simulink model "commhdlQPSKTxRxLoopback"  (R2025b)
settings: Solver=FixedStepDiscrete  StartTime=0.0  StopTime=0.03  RelTol=1e-3
PostLoadFcn:
  | hScopeConfig = get_param([gcs '/Receiver/QPSK Rx/Frequency and Time Synchronizer/Symbol Synchronizer/No HDL/QPSK Receiver Eye Diagram'],'ScopeConfiguration');
  | 
  | hScopeConfig.OpenAtSimulationStart = false;
  | hScopeConfig.Visible = false;
  | SamplesPerSymbol = 4;
  | %UpsamplesRx = 1;
  | clear hScopeConfig
InitFcn:
  | % RxAlign decoder latency (flat_simfix): 41 = netlist value used for HDL; set
  | % rxAlignLat = 25 in the base workspace before a model-level simulation.
  | if ~exist('rxAlignLat','var'), rxAlignLat = uint16(41); end
  | commhdlQPSKTxRxModelInit;
  | % Rate bridge: ADRV9002/Jupiter radio runs at 15.36 MHz = 2x the 7.68 MHz
  | % (4 samples/symbol @ Rsym=1.92 MHz) the QPSK Rx requires. The deployed
  | % Receiver must downsample the ADC stream by 2. UpsamplesRx=1 fed the QPSK
  | % Rx 8 sps (2x-upsampled) and broke symbol sync / the loopback bit check.
  | UpsamplesRx = 1;   %% T8 RATE FIX: rail 15.36e6 == ADC bus rate,
  | %% no ingress decimation (was 2 when the rail sat on the 7.68e6 rung)
  | UpsamplesTx = 1;
  | clear simTimingOffset;
StopFcn:
  | if exist('simTimingOffset','var')
  |   disp('Simulation completed');
  |   %QPSKTxRxVerification;
  | end
undefined symbols (not defined in the file or in its folder): Add, Config, fsym, randsrc, RandStream, Rsym, rxAlignLat, Shift
libraries: hdlsllib x141, simulink x45, dspsigops x30, dsphdlfiltering2 x6, dsphdlsigops2 x4, dsphdlmathfun2 x4, commdigbbndpm3 x4, dspmlti4 x2, commchan3 x1, commrflib2 x1, commcnvcod2 x1
(part 3 of 9)

== system commhdlQPSKTxRxLoopback/Transmitter/Input Data/Message Generator ==
  reset : Inport
  enable : Inport  Port=2
  MATLAB Function : MATLAB Function  TreatAsAtomicUnit=on
  out : Outport
  stop : Outport  Port=2
  start : Outport  Port=3
  valid : Outport  Port=4
  count : Outport  Port=5
  msg_count_out : Outport  Port=6
  wires:
  MATLAB Function/3(stop) -> stop/1
  MATLAB Function/1(out) -> out/1
  reset/1 -> MATLAB Function/2(reset)
  MATLAB Function/2(start) -> start/1
  enable/1 -> MATLAB Function/1(enable)
  MATLAB Function/4(valid) -> valid/1
  MATLAB Function/5(count_out) -> count/1
  MATLAB Function/6(msg_count_out) -> msg_count_out/1

== system commhdlQPSKTxRxLoopback/Transmitter/QPSK Tx/Bit Packetizer ==
  dataIn : Inport
  validIn : Inport  Port=2
  Compare To Constant : hdlsllib/Logic and Bit Operations/Compare To Constant  relop===  const=length(Preamble)  OutDataTypeStr=boolean
  Compare To Constant1 : hdlsllib/Logic and Bit Operations/Compare To Constant  relop===  const=bitsPerPacket - 1  OutDataTypeStr=boolean
  Compare To Constant2 : hdlsllib/Logic and Bit Operations/Compare To Constant  relop=>=  const=length(Preamble)  OutDataTypeStr=boolean
  Data Bits FIFO : Subsystem
  Data Type Conversion : DataTypeConversion  OutDataTypeStr=boolean  SaturateOnIntegerOverflow=off  RndMeth=Floor
  DataReadyPaceCmp : simulink/Logic and Bit Operations/Compare To Constant  relop=>=  const=SamplesPerSymbol/2 - 1  OutDataTypeStr=boolean
  HDL Counter : hdlsllib/Sources/HDL Counter  CountType=Count limited  CountInit=0  CountStep=1  CountMax=max(1, SamplesPerSymbol/2 - 1)  CountFromType=Initial value  CountFrom=0  CountResetPort=off  CountLoadPort=off  CountEnbPort=on  CountDirPort=off  CountHitOutputPort=off  CountDataType=Unsigned  CountWordLen=max(1, nextpow2(SamplesPerSymbol/2))  CountFracLen=0  CountSampTime=1
  Logical Operator : Logic  AllPortsSameDT=off  OutDataTypeStr=boolean
  Logical Operator1 : Logic  AllPortsSameDT=off  OutDataTypeStr=boolean
  Logical Operator2 : Logic  Operator=NOT  AllPortsSameDT=off  OutDataTypeStr=boolean
  Preamble Bits Generator : Subsystem
  Switch : Switch  Criteria=u2 ~= 0  SaturateOnIntegerOverflow=off  InputSameDT=off
  bitsOut : Outport
  dataStart : Outport  Port=2
  dataEnd : Outport  Port=3
  bitsValid : Outport  Port=4
  dataReady : Outport  Port=5
  wires:
  dataIn/1 -> Data Bits FIFO/1(data)
  validIn/1 -> Data Bits FIFO/2(push)
  Compare To Constant/1 -> Logical Operator/1
  Compare To Constant1/1 -> Logical Operator1/2
  Logical Operator/1 -> dataStart/1
  Logical Operator1/1 -> dataEnd/1
  Data Bits FIFO/5(fullRAM) -> Logical Operator2/1
  Logical Operator2/1 -> HDL Counter/1
  Data Bits FIFO/1(dataOut) -> Switch/1
  Data Bits FIFO/3(sampleCount) -> Preamble Bits Generator/2(sampleCount), Compare To Constant/1, Compare To Constant1/1, Compare To Constant2/1
  Data Bits FIFO/4(sampleCountValid) -> bitsValid/1, Logical Operator/2, Logical Operator1/1, Preamble Bits Generator/3(sampleCountValid)
  Data Bits FIFO/2(activeFrame) -> Preamble Bits Generator/1(activeFrame)
  Preamble Bits Generator/1(preambleBits) -> Switch/3
  Compare To Constant2/1 -> Switch/2
  Switch/1 -> bitsOut/1
  Data Type Conversion/1 -> dataReady/1
  HDL Counter/1 -> DataReadyPaceCmp/1
  DataReadyPaceCmp/1 -> Data Type Conversion/1

== system commhdlQPSKTxRxLoopback/Transmitter/QPSK Tx/HDL Data Scrambler ==
  note: HDL Data Scrambler
      | Polynomial: x^7+x^4+1
      | Initial state: [1 0 1 1 1 0 1]
  dataIn : Inport
  startIn : Inport  Port=2
  endIn : Inport  Port=3
  validIn : Inport  Port=4
  BIT_XOR : Logic  Operator=XOR  IconShape=distinctive  AllPortsSameDT=off  OutDataTypeStr=boolean
  BIT_XOR2 : Logic  Operator=XOR  IconShape=distinctive  AllPortsSameDT=off  OutDataTypeStr=boolean
  Delay{,1,3..4} (4 alike) : Delay  DelayLength=1
  EnableScrambling : Constant  Value=true  SampleTime=-1
  Logical Operator : Logic  IconShape=distinctive  AllPortsSameDT=off  OutDataTypeStr=boolean
  Switch : Switch  Criteria=u2 > Threshold  SaturateOnIntegerOverflow=off  InputSameDT=off
  Unit Delay Enabled Resettable Synchronous{,2..3,5,7} (5 alike) : hdlsllib/Discrete/Unit Delay Enabled Resettable Synchronous  InitialCondition=1  SampleTime=-1
  Unit Delay Enabled Resettable Synchronous1 : hdlsllib/Discrete/Unit Delay Enabled Resettable Synchronous  InitialCondition=0  SampleTime=-1
  Unit Delay Enabled Resettable Synchronous4 : hdlsllib/Discrete/Unit Delay Enabled Resettable Synchronous  InitialCondition=0  SampleTime=-1
  Unit Delay Enabled Resettable Synchronous6 : hdlsllib/Discrete/Unit Delay Enabled Resettable Synchronous  InitialCondition=0.0  SampleTime=-1
  dataOut : Outport  InitialOutput=0
  validOut : Outport  Port=2  InitialOutput=0
  wires:
  Delay4/1 -> validOut/1
  Delay3/1 -> dataOut/1
  endIn/1 -> Unit Delay Enabled Resettable Synchronous4/3
  Logical Operator/1 -> BIT_XOR2/2
  Unit Delay Enabled Resettable Synchronous4/1 -> Logical Operator/1
  Delay1/1 -> Unit Delay Enabled Resettable Synchronous6/2, Unit Delay Enabled Resettable Synchronous2/2, Unit Delay Enabled Resettable Synchronous1/2, Unit Delay Enabled Resettable Synchronous/2, Delay4/1, Unit Delay Enabled Resettable Synchronous3/2, Unit Delay Enabled Resettable Synchronous5/2, Unit Delay Enabled Resettable Synchronous7/2
  Delay/1 -> Switch/3, BIT_XOR2/1
  startIn/1 -> Unit Delay Enabled Resettable Synchronous4/1, Unit Delay Enabled Resettable Synchronous4/2, Unit Delay Enabled Resettable Synchronous6/3, Unit Delay Enabled Resettable Synchronous5/3, Unit Delay Enabled Resettable Synchronous1/3, Unit Delay Enabled Resettable Synchronous/3, Unit Delay Enabled Resettable Synchronous2/3, Unit Delay Enabled Resettable Synchronous3/3, Unit Delay Enabled Resettable Synchronous7/3
  dataIn/1 -> Delay/1
  validIn/1 -> Delay1/1
  BIT_XOR/1 -> Unit Delay Enabled Resettable Synchronous/1, Logical Operator/2
  Unit Delay Enabled Resettable Synchronous1/1 -> Unit Delay Enabled Resettable Synchronous2/1
  Unit Delay Enabled Resettable Synchronous2/1 -> Unit Delay Enabled Resettable Synchronous3/1
  Unit Delay Enabled Resettable Synchronous/1 -> Unit Delay Enabled Resettable Synchronous1/1
  Unit Delay Enabled Resettable Synchronous3/1 -> BIT_XOR/2, Unit Delay Enabled Resettable Synchronous5/1
  Unit Delay Enabled Resettable Synchronous5/1 -> Unit Delay Enabled Resettable Synchronous6/1
  Unit Delay Enabled Resettable Synchronous6/1 -> Unit Delay Enabled Resettable Synchronous7/1
  Unit Delay Enabled Resettable Synchronous7/1 -> BIT_XOR/1
  Switch/1 -> Delay3/1
  EnableScrambling/1 -> Switch/2
  BIT_XOR2/1 -> Switch/1

== system commhdlQPSKTxRxLoopback/Transmitter/QPSK Tx/QPSK Modulator ==
  dataIn : Inport
  validIn : Inport  Port=2
  Compare To Constant : simulink/Logic and Bit Operations/Compare To Constant  relop===  const=0  OutDataTypeStr=boolean
  Compare To Constant1 : simulink/Logic and Bit Operations/Compare To Constant  relop===  const=1  OutDataTypeStr=boolean
  Delay{,1..5,11..12} (8 alike) : Delay  DelayLength=1
  HDL Counter : hdlsllib/Sources/HDL Counter  CountType=Count limited  CountInit=0  CountStep=1  CountMax=1  CountFromType=Initial value  CountFrom=0  CountResetPort=off  CountLoadPort=off  CountEnbPort=on  CountDirPort=off  CountHitOutputPort=off  CountDataType=Unsigned  CountWordLen=1  CountFracLen=0  CountSampTime=1
  Logical Operator : Logic  IconShape=distinctive  AllPortsSameDT=off  OutDataTypeStr=boolean
  Logical Operator1 : Logic  IconShape=distinctive  AllPortsSameDT=off  OutDataTypeStr=boolean
  Mux : Mux  Inputs=2
  Null : Constant  Value=complex(0,0)  OutDataTypeStr=fixdt(1,16,15)  SampleTime=1/(Rsym*SamplesPerSymbol)
  QPSK Modulator Baseband : commdigbbndpm3/QPSK Modulator Baseband  InType=Bit  Enc=Gray  Ph=pi/4  outDtype=Fixed-point  outWordLen=16  outUDDataType=sfix(16)  outFracLenMode=User-defined  outFracLen=15  outDataTypeStr=fixdt(1,16,15)  outLastDataTypeStr=fixdt(1,16,15)
  Switch3 : Switch  Threshold=1  SaturateOnIntegerOverflow=off  InputSameDT=off
  Unit Delay Enabled Synchronous : hdlsllib/Discrete/Unit Delay Enabled Synchronous  InitialCondition=0.0  SampleTime=-1
  dataOut : Outport
  validOut : Outport  Port=2
  wires:
  dataIn/1 -> Delay/1
  validIn/1 -> Delay1/1
  HDL Counter/1 -> Compare To Constant/1, Compare To Constant1/1
  QPSK Modulator Baseband/1 -> Delay11/1
  Logical Operator1/1 -> Delay5/1
  Switch3/1 -> Delay2/1
  Null/1 -> Switch3/3
  Delay/1 -> Mux/2, Unit Delay Enabled Synchronous/1
  Delay2/1 -> dataOut/1
  Delay3/1 -> validOut/1
  Delay1/1 -> Logical Operator1/2, Logical Operator/1, HDL Counter/1
  Compare To Constant/1 -> Logical Operator/2
  Compare To Constant1/1 -> Logical Operator1/1
  Delay11/1 -> Switch3/1
  Delay12/1 -> Switch3/2, Delay3/1
  Logical Operator/1 -> Unit Delay Enabled Synchronous/2
  Unit Delay Enabled Synchronous/1 -> Mux/1
  Mux/1 -> Delay4/1
  Delay4/1 -> QPSK Modulator Baseband/1
  Delay5/1 -> Delay12/1

== system commhdlQPSKTxRxLoopback/Transmitter/QPSK Tx/RRC Transmit Filter ==
  dataIn : Inport
  validIn : Inport  Port=2
  Data Type Conversion : DataTypeConversion  OutDataTypeStr=fixdt(1,17,16)  SaturateOnIntegerOverflow=off  RndMeth=Floor
  Data Type Conversion1 : DataTypeConversion  OutDataTypeStr=fixdt(1,16,14)  SaturateOnIntegerOverflow=off  RndMeth=Floor
  Delay1 : Delay  DelayLength=1
  Delay2 : Delay  DelayLength=1
  Delay3 : Delay  DelayLength=1
  RRC Filter : dsphdlfiltering2/Discrete FIR Filter  NumeratorSource=Property  Numerator=RRCCoef  NumeratorPrototype=[]  FilterStructure=Direct form systolic  SerializationOption=Minimum number of cycles between valid input samples  NumCycles=2  NumberOfMultipliers=2  SimulateUsing=Code generation  roundingMode=Floor  overflowMode=off  CoefficientsDataTypeStr=Inherit: Same word length as input  OutputDataTypeStr=Inherit: Same word length as input  ResetInputPort=off  HDLGlobalReset=off  CoeffMultiplier=Multiplier  UseMultForPow2Coeff=on  FrameInputSymmOptim=off
  Unit Delay Enabled Synchronous1 : hdlsllib/Discrete/Unit Delay Enabled Synchronous  InitialCondition=0  SampleTime=-1
  dataOut : Outport
  validOut : Outport  Port=2
  wires:
  dataIn/1 -> Data Type Conversion/1
  RRC Filter/1 -> Data Type Conversion1/1
  RRC Filter/2 -> Delay2/1
  Delay1/1 -> dataOut/1
  Delay2/1 -> validOut/1
  Data Type Conversion/1 -> Delay3/1
  Unit Delay Enabled Synchronous1/1 -> RRC Filter/2
  Data Type Conversion1/1 -> Delay1/1
  validIn/1 -> Unit Delay Enabled Synchronous1/2, Unit Delay Enabled Synchronous1/1
  Delay3/1 -> RRC Filter/1

== system commhdlQPSKTxRxLoopback/TxRxComposite/Receiver/Capture Data Bits ==
  dataOut : Inport
  dataSrt : Inport  Port=2
  dataEnd : Inport  Port=3
  valid : Inport  Port=4
  Display : Display
  Display1 : Display
  Display2 : Display
  MATLAB Function : MATLAB Function  TreatAsAtomicUnit=on
  count_out : Outport
  packets_out : Outport  Port=2
  bit_errors_out : Outport  Port=3
  wires:
  MATLAB Function/3(bit_errors_out) -> bit_errors_out/1, Display2/1
  MATLAB Function/2(packets_out) -> packets_out/1, Display1/1
  valid/1 -> MATLAB Function/1(valid)
  dataSrt/1 -> MATLAB Function/3(start)
  MATLAB Function/1(count_out) -> count_out/1, Display/1
  dataEnd/1 -> MATLAB Function/4(stop)
  dataOut/1 -> MATLAB Function/2(datain)

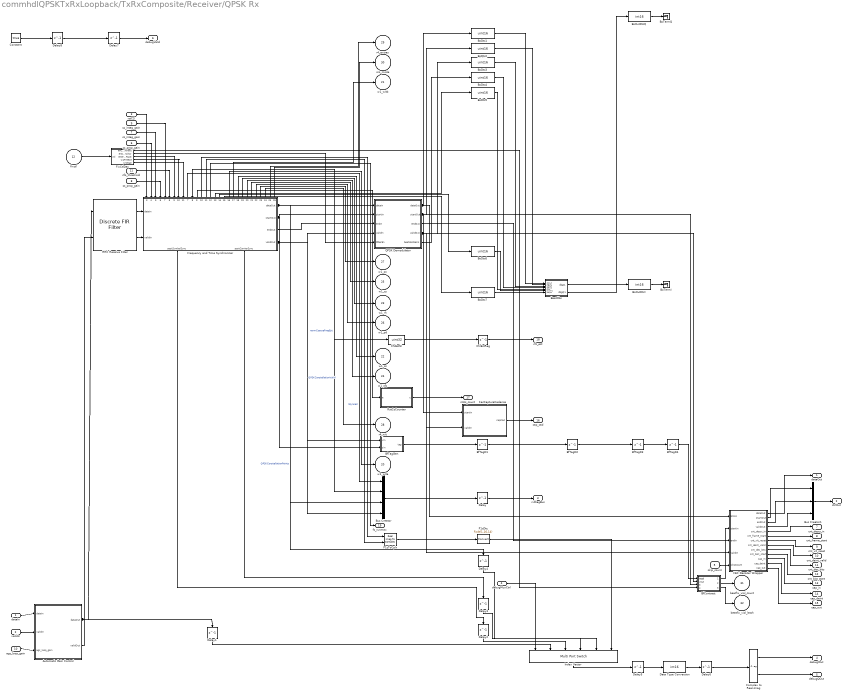
== system commhdlQPSKTxRxLoopback/TxRxComposite/Receiver/QPSK Rx ==
  dataIn : Inport  OutDataTypeStr=fixdt(1,16,14)  PortDimensions=1  SampleTime=1/(Rsym*SamplesPerSymbol)
      settings: SignalType=complex
  validIn : Inport  Port=2  OutDataTypeStr=boolean  PortDimensions=1  SampleTime=1/(Rsym*SamplesPerSymbol)
  rstCS : Inport  Port=3  OutDataTypeStr=boolean  PortDimensions=1
      settings: SignalType=complex
  debugMuxCtrl : Inport  Port=4  OutDataTypeStr=uint32  PortDimensions=1  SampleTime=1/(Rsym*SamplesPerSymbol)
  skip_count : Inport  Port=5  OutDataTypeStr=uint32  SampleTime=1/(Rsym*SamplesPerSymbol)
  cs_prop_gain : Inport  Port=6  OutDataTypeStr=uint32  SampleTime=1/(Rsym*SamplesPerSymbol)
  cs_integ_gain : Inport  Port=7  OutDataTypeStr=uint32  SampleTime=1/(Rsym*SamplesPerSymbol)
  ss_prop_gain : Inport  Port=8  OutDataTypeStr=uint32  SampleTime=1/(Rsym*SamplesPerSymbol)
  ss_integ_gain : Inport  Port=9  OutDataTypeStr=uint32  SampleTime=1/(Rsym*SamplesPerSymbol)
  agc_loop_gain : Inport  Port=10  OutDataTypeStr=uint32  SampleTime=1/(Rsym*SamplesPerSymbol)
  cfo_threshold : Inport  Port=11  OutDataTypeStr=uint32  SampleTime=1/(Rsym*SamplesPerSymbol)
  fixctl : Inport  Port=12  OutDataTypeStr=uint32
  Automatic Gain Control : Subsystem  mask{Ref=AGCReference, LFG=AGCLoopGain}
      mask prompts: Ref "Error Detector Reference:"; LFG "Loop Filter Gain"
  BeatObs : MATLAB Function  TreatAsAtomicUnit=on
  BfContract : MATLAB Function  TreatAsAtomicUnit=on
  BfTagD{1..4} (4 alike) : Delay  DelayLength=1
  BfTagGen : MATLAB Function  TreatAsAtomicUnit=on
  BoDtc{1..7} (7 alike) : DataTypeConversion  OutDataTypeStr=uint16  ConvertRealWorld=Stored Integer (SI)  SaturateOnIntegerOverflow=off  RndMeth=Floor
  BoOutDtcI : DataTypeConversion  OutDataTypeStr=int16  ConvertRealWorld=Stored Integer (SI)  SaturateOnIntegerOverflow=off  RndMeth=Floor
  BoOutDtcQ : DataTypeConversion  OutDataTypeStr=int16  ConvertRealWorld=Stored Integer (SI)  SaturateOnIntegerOverflow=off  RndMeth=Floor
  BoTermI : Terminator
  BoTermQ : Terminator
  Bus Creator : BusCreator  Inputs=4
  Bus Creator1 : BusCreator  Inputs=3
  CfcEstReg : Delay  DelayLength=1
  CfcEstSI : DataTypeConversion  OutDataTypeStr=uint32  ConvertRealWorld=Stored Integer (SI)
  Complex to Real-Imag : ComplexToRealImag
  Constant : Constant  Value=true  SampleTime=1/(Rsym*SamplesPerSymbol)
  Data Type Conversion : DataTypeConversion  OutDataTypeStr=int16  ConvertRealWorld=Stored Integer (SI)  SaturateOnIntegerOverflow=off  RndMeth=Floor
  Delay{,1..8} (9 alike) : Delay  DelayLength=1
  FEC Decoder Wrapper : Subsystem
  FecCaptureCadence : MATLAB Function  TreatAsAtomicUnit=on
  FixCtlDec : MATLAB Function  TreatAsAtomicUnit=on
  Frequency and Time Synchronizer : Subsystem
      settings: PortSchema="{\"entries\":[{\"content\":{\"sides\":[{\"content\":{\"connectorIds\":[\"In1\",\"In2\"]},\"type\":\"ConnectorPlacement.EquallySpacedRectSide\",\"uuid\":\"8bc6a452-5111-4806-8ca9-335cb622aea6\"},{\"content\":{\"connectorIds\":[\"Out1\",\"Out2\",\"Out3\",\"Out4\"],\"side\":\"RIGHT\"},\"type\":\"ConnectorPlacement.EquallySpacedRectSide\",\"uuid\":\"b0f43c98-f5c0-4f62-94ae-d69789942eef\"},{\"content\":{\"connectorIds\":[\"In3\",\"In4\",\"In5\",\"In6\",\"In7\",\"In8\",\"In9\",\"In10\",\"In11\",\"Out7\",\"Out8\",\"Out9\",\"Out10\",\"Out11\",\"Out12\",\"Out13\",\"Out14\",\"Out15\",\"Out16\",\"Out17\",\"Out18\",\"Out19\",\"Out20\",\"Out21\",\"Out22\",\"Out23\",\"Out24\",\"Out25\",\"Out26\"],\"side\":\"TOP\"},\"type\":\"ConnectorPlacement.EquallySpacedRectSide\",\"uuid\":\"427ff3b3-b896-4008-9584-d311480df763\"},{\"content\":{\"connectorIds\":[\"Out5\",\"Out6\"],\"side\":\"BOTTOM\"},\"type\":\"ConnectorPlacement.EquallySpacedRectSide\",\"uuid\":\"f704cb90-80a1-4198-8b72-e70182b45e73\"},{\"content\":{\"side\":\"HIDDEN\"},\"type\":\"ConnectorPlacement.EquallySpacedRectSide\",\"uuid\":\"f6309498-1e43-486f-b6b5-2c6570711f8e\"}]},\"type\":\"ConnectorPlacement.EquallySpacedConnector\",\"uuid\":\"f0ce492e-c9e1-4b35-98ef-84d77b696cfe\"}],\"packageUris\":[\"http://schema.mathworks.com/mf0/Connector/R2020b\"],\"version\":\"1.0\"}"
  Index Vector : MultiPortSwitch  DataPortOrder=Zero-based contiguous  Inputs=5  DiagnosticForDefault=None  zeroidx=on  SaturateOnIntegerOverflow=off  InputSameDT=off
  P1cDtc : DataTypeConversion  OutDataTypeStr=fixdt(1,16,14)  ConvertRealWorld=Stored Integer (SI)  SaturateOnIntegerOverflow=off  RndMeth=Floor
  P1cToCplx : RealImagToComplex
  QPSK Demodulator : Subsystem
  RRC Receive Filter : dsphdlfiltering2/Discrete FIR Filter  NumeratorSource=Property  Numerator=RRCCoef  NumeratorPrototype=[]  FilterStructure=Direct form systolic  SerializationOption=Minimum number of cycles between valid input samples  NumCycles=2  NumberOfMultipliers=2  SimulateUsing=Code generation  roundingMode=Floor  overflowMode=off  CoefficientsDataTypeStr=Inherit: Same word length as input  OutputDataTypeStr=Inherit: Same word length as input  ResetInputPort=off  HDLGlobalReset=off  CoeffMultiplier=Multiplier  UseMultForPow2Coeff=on  FrameInputSymmOptim=off
  RstCsCounter : MATLAB Function  TreatAsAtomicUnit=on
  dataOut : Outport
  ctrlOut : Outport  Port=2
  rxDiagBus : Outport  Port=3
  debugIOut : Outport  Port=4
  debugQOut : Outport  Port=5
  debugValid : Outport  Port=6
  cnt_descr_in : Outport  Port=7
  cnt_frame_start : Outport  Port=8
  cnt_vit_reset : Outport  Port=9
  cnt_deint_valid : Outport  Port=10
  cnt_dec_bits : Outport  Port=11
  cnt_bist_start : Outport  Port=12
  cap_in : Outport  Port=13
  cap_deint : Outport  Port=14
  cap_out : Outport  Port=15
  cap_cad : Outport  Port=16
  rstcs_count : Outport  Port=17
  cfc_est : Outport  Port=18
  fs_runmax : Outport  Port=19
  w1_wita : Outport  Port=20
  w1_witb : Outport  Port=21
  w1_ss : Outport  Port=22
  w1_rh : Outport  Port=23
  w1_cfc : Outport  Port=24
  w1_cs : Outport  Port=25
  w1_pd : Outport  Port=26
  w1_pc : Outport  Port=27
  r4_wit : Outport  Port=28
  r4_extras : Outport  Port=29
  sro_mode : Outport  Port=30
  beatfix_viol_count : Outport  Port=31
  beatfix_viol_latch : Outport  Port=32
  wires:
  Bus Creator1/1 -> ctrlOut/1
  FEC Decoder Wrapper/10(cnt_bist_start) -> cnt_bist_start/1
  FEC Decoder Wrapper/8(cnt_deint_valid) -> cnt_deint_valid/1
  FEC Decoder Wrapper/7(cnt_vit_reset) -> cnt_vit_reset/1
  FEC Decoder Wrapper/5(cnt_descr_in) -> cnt_descr_in/1
  Complex to Real-Imag/2 -> debugQOut/1
  FEC Decoder Wrapper/3(endOut) -> Bus Creator1/2
  FEC Decoder Wrapper/9(cnt_dec_bits) -> cnt_dec_bits/1
  skip_count/1 -> FEC Decoder Wrapper/5(skipCount)
  Delay5/1 -> Data Type Conversion/1
  BoOutDtcI/1 -> BoTermI/1
  BfTagD2/1 -> BfTagD3/1
  debugMuxCtrl/1 -> Index Vector/1
  P1cDtc/1 -> Index Vector/6
  BfTagD1/1 -> BfTagD2/1
  FecCaptureCadence/1(capCad) -> cap_cad/1
  BoDtc7/1 -> BeatObs/7(popc)
  BoDtc6/1 -> BeatObs/6(pushc)
  BoDtc3/1 -> BeatObs/3(vOut)
  BoDtc2/1 -> BeatObs/2(sOut)
  BoDtc1/1 -> BeatObs/1(dOut)
  Delay2/1 -> Index Vector/3
  Delay4/1 -> Index Vector/5
  Frequency and Time Synchronizer/6(postCarrierSync) -> Delay3/1
  Frequency and Time Synchronizer/10(p1c_telI) -> P1cToCplx/1
  FEC Decoder Wrapper/2(startOut) -> Bus Creator1/1
  RRC Receive Filter/1 -> Frequency and Time Synchronizer/1(dataIn)
  Frequency and Time Synchronizer/5(postSymbolSync) -> Delay2/1
  BfContract/3(violLatch) -> beatfix_viol_latch/1
  Frequency and Time Synchronizer/8(normCoarseFreqEst) -> Bus Creator/2, CfcEstSI/1  "normCoarseFreqEst"
  Frequency and Time Synchronizer/21(w1_cs) -> w1_cs/1
  cfo_threshold/1 -> Frequency and Time Synchronizer/8(cfo_threshold)
  Frequency and Time Synchronizer/13(beatobsRhCtr) -> BoDtc5/1
  BfContract/1(startSel) -> FEC Decoder Wrapper/2(startIn)
  Index Vector/1 -> Delay5/1
  FixCtlDec/5(sroSign) -> Frequency and Time Synchronizer/11(sroSign)
  BfContract/2(violCount) -> beatfix_viol_count/1
  QPSK Demodulator/3(endOut) -> FEC Decoder Wrapper/3(endIn)
  FixCtlDec/4(w1Freeze) -> Frequency and Time Synchronizer/10(w1Freeze)
  Frequency and Time Synchronizer/3(endOut) -> QPSK Demodulator/3(endIn)
  agc_loop_gain/1 -> Automatic Gain Control/3(agc_loop_gain)
  Frequency and Time Synchronizer/23(w1_pc) -> w1_pc/1
  Automatic Gain Control/2(validOut) -> RRC Receive Filter/2
  Frequency and Time Synchronizer/24(r4_wit) -> r4_wit/1
  BfTagD3/1 -> BfTagD4/1
  BeatObs/1(dbgI1) -> BoOutDtcI/1
  BoDtc5/1 -> BeatObs/5(rhc)
  Delay1/1 -> Index Vector/2
  Data Type Conversion/1 -> Delay6/1
  Frequency and Time Synchronizer/12(fs_runmax) -> fs_runmax/1
  ss_prop_gain/1 -> Frequency and Time Synchronizer/6(ss_prop_gain)
  RRC Receive Filter/2 -> Frequency and Time Synchronizer/2(validIn)
  Frequency and Time Synchronizer/26(sro_mode) -> sro_mode/1
  FixCtlDec/2(enSerAnchor) -> QPSK Demodulator/5(bfSerEn)
  cs_prop_gain/1 -> Frequency and Time Synchronizer/4(cs_prop_gain)
  FEC Decoder Wrapper/13(cap_out) -> cap_out/1
  BoDtc4/1 -> BeatObs/4(decis)
  Constant/1 -> Delay8/1
  cs_integ_gain/1 -> Frequency and Time Synchronizer/5(cs_integ_gain)
  FixCtlDec/3(enGridPace) -> Frequency and Time Synchronizer/9(bfGridEn)
  QPSK Demodulator/1(dataOut) -> BoDtc1/1, FEC Decoder Wrapper/1(bitsIn)
  FixCtlDec/1(enContract) -> BfContract/4(enContract)
  CfcEstReg/1 -> cfc_est/1
  fixctl/1 -> FixCtlDec/1(ctl)
  dataIn/1 -> Automatic Gain Control/1(dataIn)
  BoOutDtcQ/1 -> BoTermQ/1
  Delay7/1 -> debugValid/1
  Frequency and Time Synchronizer/11(p1c_telQ) -> P1cToCplx/2
  Automatic Gain Control/1(dataOut) -> RRC Receive Filter/1, Delay1/1
  FEC Decoder Wrapper/1(dataOut) -> dataOut/1
  Frequency and Time Synchronizer/1(dataOut) -> Bus Creator/3, QPSK Demodulator/1(dataIn), Delay4/1  "QPSKConstellationPoints"
  Frequency and Time Synchronizer/2(startOut) -> BfTagGen/2(sin), QPSK Demodulator/2(startIn)
  rstCS/1 -> Frequency and Time Synchronizer/3(rstCS)
  Complex to Real-Imag/1 -> debugIOut/1
  FEC Decoder Wrapper/12(cap_deint) -> cap_deint/1
  ss_integ_gain/1 -> Frequency and Time Synchronizer/7(ss_integ_gain)
  BfTagD4/1 -> BfContract/1(tagd)
  Delay8/1 -> Delay7/1
  Frequency and Time Synchronizer/9(rstcsDet) -> RstCsCounter/1(e)
  Frequency and Time Synchronizer/4(validOut) -> BfTagGen/1(vin), QPSK Demodulator/4(validIn), Bus Creator/4  "QPSKConstellationValid"
  validIn/1 -> Automatic Gain Control/2(validIn)
  Frequency and Time Synchronizer/14(beatobsPush) -> BoDtc6/1
  Frequency and Time Synchronizer/15(beatobsPop) -> BoDtc7/1
  FEC Decoder Wrapper/11(cap_in) -> cap_in/1
  Frequency and Time Synchronizer/16(w1_wita) -> w1_wita/1
  Frequency and Time Synchronizer/22(w1_pd) -> w1_pd/1
  CfcEstSI/1 -> CfcEstReg/1
  Frequency and Time Synchronizer/17(w1_witb) -> w1_witb/1
  Frequency and Time Synchronizer/18(w1_ss) -> w1_ss/1
  Frequency and Time Synchronizer/19(w1_rh) -> w1_rh/1
  Frequency and Time Synchronizer/20(w1_cfc) -> w1_cfc/1
  Frequency and Time Synchronizer/25(r4_extras) -> r4_extras/1
  FEC Decoder Wrapper/4(validOut) -> Bus Creator1/3
  BeatObs/2(dbgQ1) -> BoOutDtcQ/1
  QPSK Demodulator/2(startOut) -> FecCaptureCadence/1(startIn), BoDtc2/1, BfContract/3(legacyStart)
  FEC Decoder Wrapper/6(cnt_frame_start) -> cnt_frame_start/1
  QPSK Demodulator/4(validOut) -> BoDtc3/1, FecCaptureCadence/2(validIn), BfContract/2(vout), FEC Decoder Wrapper/4(validIn)
  QPSK Demodulator/5(beatobsDecis) -> BoDtc4/1
  RstCsCounter/1(c) -> rstcs_count/1
  BfTagGen/1(tag) -> BfTagD1/1
  Delay6/1 -> Complex to Real-Imag/1
  Delay/1 -> rxDiagBus/1
  Bus Creator/1 -> Delay/1
  Delay3/1 -> Index Vector/4
  Frequency and Time Synchronizer/7(nSynced) -> Bus Creator/1  "nSynced"
  P1cToCplx/1 -> P1cDtc/1

== system commhdlQPSKTxRxLoopback/TxRxComposite/Transmitter/Input Data ==
  enb : Inport
  reset : Inport  Port=2
  extWord : Inport  Port=3  OutDataTypeStr=uint64
  extWordAvail : Inport  Port=4  OutDataTypeStr=boolean
  extBitSel : Inport  Port=5  OutDataTypeStr=boolean
  extWordFirst : Inport  Port=6  OutDataTypeStr=boolean
  BitMux : Switch  Criteria=u2 ~= 0
  ByteBitShifter : MATLAB Function  TreatAsAtomicUnit=on
  Cast To Boolean : DataTypeConversion  OutDataTypeStr=boolean  SaturateOnIntegerOverflow=off  RndMeth=Floor
  Delay : Delay  DelayLength=1
  Display : Display
  FEC Tx Encoder K5 : Subsystem
  Message Generator : Subsystem
  Terminator : Terminator
  Terminator1 : Terminator
  txData : Outport
  txValid : Outport  Port=2
  msg_count_out : Outport  Port=3
  extWordPop : Outport  Port=4
  fs_txur : Outport  Port=5
  wires:
  BitMux/1 -> txData/1
  extBitSel/1 -> BitMux/2
  ByteBitShifter/3(txur) -> fs_txur/1
  ByteBitShifter/2(popToggle) -> extWordPop/1
  Cast To Boolean/1 -> FEC Tx Encoder K5/3(reset), ByteBitShifter/2(reset), Message Generator/1(reset)
  reset/1 -> Terminator/1
  Message Generator/1(out) -> BitMux/3
  enb/1 -> Message Generator/2(enable), FEC Tx Encoder K5/2(enable), ByteBitShifter/1(enable)
  Message Generator/4(valid) -> txValid/1
  FEC Tx Encoder K5/1(encBit) -> BitMux/1
  extWord/1 -> ByteBitShifter/4(extWord)
  Message Generator/2(stop) -> Delay/1
  ByteBitShifter/1(bit) -> FEC Tx Encoder K5/1(bitIn)
  Message Generator/3(start) -> ByteBitShifter/3(start), Terminator1/1, FEC Tx Encoder K5/4(start)
  Delay/1 -> Cast To Boolean/1
  Message Generator/5(count) -> Display/1
  Message Generator/6(msg_count_out) -> msg_count_out/1
  extWordAvail/1 -> ByteBitShifter/5(extWordAvail)
  extWordFirst/1 -> ByteBitShifter/6(extWordFirst)

== system commhdlQPSKTxRxLoopback/TxRxComposite/Transmitter/QPSK Tx ==
  dataIn : Inport  OutDataTypeStr=boolean  PortDimensions=1
  validIn : Inport  Port=2  OutDataTypeStr=boolean  PortDimensions=1
  Bit Packetizer : Subsystem
  Bus Creator : BusCreator  Inputs=2
  HDL Data Scrambler : Subsystem
  QPSK Modulator : Subsystem
  RRC Transmit Filter : Subsystem
  dataReady : Outport
  dataOut : Outport  Port=2
  txDiagBus : Outport  Port=3
  validOut : Outport  Port=4
  wires:
  validIn/1 -> Bit Packetizer/2(validIn)
  Bit Packetizer/1(bitsOut) -> HDL Data Scrambler/1(dataIn)
  Bit Packetizer/4(bitsValid) -> HDL Data Scrambler/4(validIn)
  QPSK Modulator/2(validOut) -> Bus Creator/2, RRC Transmit Filter/2(validIn)  "QPSKConstellationValid"
  dataIn/1 -> Bit Packetizer/1(dataIn)
  Bit Packetizer/2(dataStart) -> HDL Data Scrambler/2(startIn)
  Bit Packetizer/3(dataEnd) -> HDL Data Scrambler/3(endIn)
  Bus Creator/1 -> txDiagBus/1
  Bit Packetizer/5(dataReady) -> dataReady/1
  HDL Data Scrambler/2(validOut) -> QPSK Modulator/2(validIn)
  QPSK Modulator/1(dataOut) -> Bus Creator/1, RRC Transmit Filter/1(dataIn)  "QPSKConstellationPoints"
  RRC Transmit Filter/1(dataOut) -> dataOut/1
  HDL Data Scrambler/1(dataOut) -> QPSK Modulator/1(dataIn)
  RRC Transmit Filter/2(validOut) -> validOut/1

== system commhdlQPSKTxRxLoopback/Receiver/QPSK Rx/Automatic Gain Control/Error Detector ==
  dataIn : Inport
  Add1 : Sum  Inputs=+-
  Conj : Math  Operator=conj
  Data Type Duplicate : DataTypeDuplicate
  Delay{,1..3} (4 alike) : Delay
  Product : Product
  Ref : Constant  Value=Ref  OutDataTypeStr=Inherit: Inherit via back propagation  SampleTime=-1
  err : Outport
  wires:
  Delay3/1 -> err/1
  Delay2/1 -> Add1/2
  Delay1/1 -> Product/1
  Delay/1 -> Product/2
  Ref/1 -> Data Type Duplicate/1, Add1/1
  Conj/1 -> Delay/1
  Product/1 -> Delay2/1
  dataIn/1 -> Conj/1, Data Type Duplicate/2, Delay1/1
  Add1/1 -> Delay3/1

== system commhdlQPSKTxRxLoopback/Receiver/QPSK Rx/Automatic Gain Control/Loop Filter ==
  note: Fixed point precision loss warnings
      | are supressed in Mask Init Callback
  err : Inport
  Add : Sum  Inputs=|++  OutDataTypeStr=Inherit: Same as first input
  Delay1 : Delay  DelayLength=1
  Delay2 : Delay
  Delay3 : Delay
  Gain1 : Gain  Gain=LFG  OutDataTypeStr=fixdt(1,34,28)
      mask init:
      | Simulink.suppressDiagnostic(gcb, 'SimulinkFixedPoint:util:fxpParameterPrecisionLoss');
  gain : Outport
  wires:
  Delay3/1 -> Gain1/1
  Delay2/1 -> Add/1
  Gain1/1 -> Delay2/1
  Add/1 -> Delay1/1
  Delay1/1 -> Add/2, gain/1
  err/1 -> Delay3/1

== system commhdlQPSKTxRxLoopback/Receiver/QPSK Rx/Frequency and Time Synchronizer/Carrier Synchronizer ==
  dataIn : Inport
  internalRst : Inport  Port=2
  validIn : Inport  Port=3
  manualRst : Inport  Port=4
  Data Type Conversion2 : DataTypeConversion  OutDataTypeStr=fixdt(1,16,14)  SaturateOnIntegerOverflow=off  RndMeth=Floor
  Delay{,2,5,7,11} (5 alike) : Delay  DelayLength=1
  Delay{1,10,14..15} (4 alike) : Delay  DelayLength=6
  Delay{3..4,6,8..9,12..13} (7 alike) : Delay
  Direct Digital Synthesis : Subsystem
  Logical Operator : Logic  AllPortsSameDT=off  OutDataTypeStr=boolean
  Loop Filter : Subsystem
  Math Function : Math  Operator=conj  SignedPower=on  RndMeth=Zero
  Phase Error Detector : Subsystem
  Product : Product
  dataOut : Outport
  validOut : Outport  Port=2
  wires:
  Delay/1 -> Phase Error Detector/1(dataIn)
  Math Function/1 -> Delay3/1
  Data Type Conversion2/1 -> Delay5/1, Delay/1
  Delay3/1 -> Product/2
  Product/1 -> Delay6/1
  Delay8/1 -> Delay2/1, Delay7/1
  Delay9/1 -> Delay8/1
  Delay4/1 -> Product/1
  Delay6/1 -> Data Type Conversion2/1
  Direct Digital Synthesis/1(expOut) -> Math Function/1
  Loop Filter/1(v) -> Direct Digital Synthesis/3(phaseInc)
  Phase Error Detector/1(PhaseError) -> Loop Filter/1(e)
  Delay2/1 -> Delay1/1
  Delay1/1 -> Loop Filter/2(validIn)
  Delay10/1 -> Delay4/1
  Delay11/1 -> Delay15/1
  Delay12/1 -> Delay11/1
  Delay13/1 -> Delay12/1
  Loop Filter/2(valid) -> Direct Digital Synthesis/2(validIn)
  Delay5/1 -> dataOut/1
  Delay7/1 -> validOut/1
  dataIn/1 -> Delay10/1
  internalRst/1 -> Delay13/1
  validIn/1 -> Delay14/1
  Delay14/1 -> Delay9/1
  manualRst/1 -> Logical Operator/1, Loop Filter/4(externalRst)
  Delay15/1 -> Loop Filter/3(internalRst)
  Loop Filter/3(rst) -> Logical Operator/2
  Logical Operator/1 -> Direct Digital Synthesis/1(rst)

== system commhdlQPSKTxRxLoopback/Receiver/QPSK Rx/Frequency and Time Synchronizer/Coarse Frequency Compensator ==
  dataIn : Inport
  validIn : Inport  Port=2
  CFO step change detector : Subsystem
  Coarse Frequency Estimator : Subsystem
  Data Type Conversion2 : DataTypeConversion  OutDataTypeStr=fixdt(1,16,12)  SaturateOnIntegerOverflow=off  RndMeth=Floor
  Data Type Conversion3 : DataTypeConversion  OutDataTypeStr=fixdt(1,21,21)  SaturateOnIntegerOverflow=off  RndMeth=Floor
  Data Type Conversion4 : DataTypeConversion  OutDataTypeStr=fixdt(1,21,0)  ConvertRealWorld=Stored Integer (SI)  SaturateOnIntegerOverflow=off  RndMeth=Floor
  Delay1 : Delay  DelayLength=9
  Delay{11..17} (7 alike) : Delay
  Delay2 : Delay  DelayLength=9
  Delay3 : Delay  DelayLength=6
  Delay4 : Delay  DelayLength=6
  Delay5 : Delay  DelayLength=1
  Delay6 : Delay  DelayLength=1
  Delay7 : Delay  DelayLength=12
  Delay8 : Delay  DelayLength=12
  Gain : Gain  Gain=1/4  ParamDataTypeStr=fixdt(0,2,2)  OutDataTypeStr=Inherit: Same as input
  Math Function : Math  Operator=conj
  NCO : dsphdlsigops2/NCO  PhaseIncrementSource=Input port  PhaseIncrement=100  PhaseOffsetSource=Property  PhaseOffset=0  DitherSource=None  NumDitherBits=4  SamplesPerFrame=1  LUTCompress=off  ResetAction=off  Waveform=Complex exponential  PhasePort=off  SimulateUsing=Code generation  AccumulatorWL=21  PhaseQuantization=on  NumQuantizerAccumulatorBits=14  OutputDataType=Binary point scaling  OutputWL=16  OutputFL=14
  Product1 : Product  OutDataTypeStr=Inherit: Same as first input
  Raise Power to 4 : Subsystem
  Terminator : Terminator
  dataOut : Outport
  rstCS : Outport  Port=2
  validOut : Outport  Port=3
  normalizedFreqEst : Outport  Port=4
  wires:
  Delay14/1 -> Delay15/1
  Delay11/1 -> Product1/1
  Delay6/1 -> Raise Power to 4/2(validIn), Delay2/1
  Delay5/1 -> Delay1/1, Data Type Conversion2/1
  Data Type Conversion4/1 -> NCO/1
  Delay4/1 -> Delay14/1
  Delay3/1 -> Delay11/1
  Delay2/1 -> Delay8/1
  Delay1/1 -> Delay7/1
  NCO/2 -> Terminator/1
  NCO/1 -> Math Function/1
  Product1/1 -> Delay13/1
  Raise Power to 4/2(validOut) -> Coarse Frequency Estimator/2(validIn)
  Math Function/1 -> Delay12/1
  Raise Power to 4/1(dataOut) -> Coarse Frequency Estimator/1(dataIn)
  Delay12/1 -> Product1/2
  Coarse Frequency Estimator/1(normFreqEst) -> Gain/1
  Data Type Conversion2/1 -> Raise Power to 4/1(dataIn)
  Delay16/1 -> Delay17/1
  CFO step change detector/1(Out1) -> Delay16/1
  Gain/1 -> Data Type Conversion3/1
  Delay13/1 -> dataOut/1
  dataIn/1 -> Delay5/1
  validIn/1 -> Delay6/1
  Delay17/1 -> rstCS/1
  Data Type Conversion3/1 -> normalizedFreqEst/1, CFO step change detector/1(In1), Data Type Conversion4/1
  Delay15/1 -> validOut/1
  Delay7/1 -> Delay3/1
  Delay8/1 -> NCO/2, Delay4/1

== system commhdlQPSKTxRxLoopback/Receiver/QPSK Rx/Frequency and Time Synchronizer/No HDL ==
  In1 : Inport
  In2 : Inport  Port=2
  In3 : Inport  Port=3
  In4 : Inport  Port=4
  Data Type Conversion : DataTypeConversion  OutDataTypeStr=double  SaturateOnIntegerOverflow=off  RndMeth=Floor
  Data Type Conversion1 : DataTypeConversion  OutDataTypeStr=double  SaturateOnIntegerOverflow=off  RndMeth=Floor
  QPSK Receiver Constellations 2 : ConstellationDiagram  NumInputPorts=2  WindowPosition=[67.000000,180.000000,973.000000,678.000000,]  Visible=on  ScopeFrameLocation=window  SymbolsToDisplaySource=Property  SymbolsToDisplay=10000  ReferenceConstellation="{[0.70711+0.70711i        -0.70711+0.70711i        -0.70711-0.70711i         0.70711-0.70711i],[0.70711+0.70711i        -0.70711+0.70711i        -0.70711-0.70711i         0.70711-0.70711i]}"  ReferenceMarker={''+'',''+''}  ReferenceColor={[1 0 0],[1 0 0]}  XLimits=[-1.3581 1.3569]  YLimits=[-1.3581 1.3569]  AxesLimits=[-1.3581 1.3569]  ShowLegend=on  DefaultConfigurationName=comm.scopes.ConstellationDiagramBlockCfg
      settings: OpenAtSimulationStart=off
  Subsystem : Subsystem
  Unit Delay Enabled Synchronous : hdlsllib/Discrete/Unit Delay Enabled Synchronous  InitialCondition=0.0  SampleTime=-1
  Unit Delay Enabled Synchronous1 : hdlsllib/Discrete/Unit Delay Enabled Synchronous  InitialCondition=0.0  SampleTime=-1
  wires:
  In4/1 -> Unit Delay Enabled Synchronous1/2, Subsystem/Enable
  Data Type Conversion/1 -> Unit Delay Enabled Synchronous1/1, Subsystem/1(In1)
  Unit Delay Enabled Synchronous1/1 -> QPSK Receiver Constellations 2/2  "After Carrier Synchronization"
  In2/1 -> Unit Delay Enabled Synchronous/2
  In1/1 -> Data Type Conversion1/1
  Data Type Conversion1/1 -> Unit Delay Enabled Synchronous/1
  Unit Delay Enabled Synchronous/1 -> QPSK Receiver Constellations 2/1  "After Symbol Synchronization"
  In3/1 -> Data Type Conversion/1

== system commhdlQPSKTxRxLoopback/Receiver/QPSK Rx/Frequency and Time Synchronizer/Packet Controller ==
  dataIn : Inport
  syncPulse : Inport  Port=2
  validIn : Inport  Port=3
  Delay : Delay  DelayLength=4
  Delay1 : Delay  DelayLength=4
  Delay2 : Delay  DelayLength=4
  End Generator : Subsystem
  Logical Operator : Logic  IconShape=distinctive  AllPortsSameDT=off  OutDataTypeStr=boolean
  MATLAB Function : MATLAB Function  TreatAsAtomicUnit=on
  Time Scope End Generator : Scope  Commented=on  NumInputPorts=2
      settings: SampleTime=1  ActiveDisplayYMinimum=-0.048155737704917989  ActiveDisplayYMaximum=1.0464480874316939  YLabel=Amplitude  DataLoggingVariableName=ScopeData2
  To File : ToFile  Filename=end_gen.mat  MatrixName=end_gen  SaveFormat=Timeseries
  To File1 : ToFile  Filename=reset  MatrixName=reset  SaveFormat=Timeseries
  sample discard controller : MATLAB Function  TreatAsAtomicUnit=on
  dataOut : Outport
  startOut : Outport  Port=2
  endOut : Outport  Port=3
  validOut : Outport  Port=4
  wires:
  MATLAB Function/1(out) -> Logical Operator/2
  sample discard controller/1(dataOut) -> dataOut/1
  sample discard controller/2(startOut) -> startOut/1
  sample discard controller/3(endOut) -> endOut/1
  sample discard controller/4(validOut) -> validOut/1
  Delay/1 -> sample discard controller/1(dataIn)
  Delay1/1 -> sample discard controller/2(validIn), End Generator/1(validIn)
  Delay2/1 -> sample discard controller/3(startIn)
  dataIn/1 -> Delay/1
  validIn/1 -> MATLAB Function/1(valid), Delay1/1, Logical Operator/1
  Logical Operator/1 -> Delay2/1, To File1/1, Time Scope End Generator/2, End Generator/2(rst)
  syncPulse/1 -> MATLAB Function/2(syncPulse)
  End Generator/1(endOut) -> Time Scope End Generator/1, To File/1, sample discard controller/4(endIn)

== system commhdlQPSKTxRxLoopback/Receiver/QPSK Rx/Frequency and Time Synchronizer/Phase Ambiguity Estimation and Correction ==
  dataIn : Inport
  syncPulseIn : Inport  Port=2
  validIn : Inport  Port=3
  Average Estimates : Subsystem
  Delay : Delay  DelayLength=32
  Delay1 : Delay  DelayLength=32
  Delay10 : Delay  DelayLength=15 + 7
  Delay11 : Delay  DelayLength=5
  Delay12 : Delay  DelayLength=5
  Delay13 : Delay  DelayLength=5
  Delay2 : Delay  DelayLength=32
  Delay3 : Delay  DelayLength=8
  Delay4 : Delay  DelayLength=8
  Delay5 : Delay  DelayLength=8
  Delay6 : Delay  DelayLength=1
  Delay7 : Delay  DelayLength=1
  Delay8 : Delay  DelayLength=1
  Delay9 : Delay  DelayLength=10
  EstDataLookback : Delay  DelayLength=6
  EstVldLookback : Delay  DelayLength=6
  Phase Ambiguity Corrector : Subsystem
  Phase Ambiguity Estimator : Subsystem
  dataOut : Outport
  syncPulseOut : Outport  Port=2
  validOut : Outport  Port=3
  wires:
  Delay4/1 -> Delay2/1
  Delay5/1 -> Delay/1
  Delay3/1 -> Delay1/1
  Delay10/1 -> Delay9/1
  Phase Ambiguity Corrector/1(dataOut) -> dataOut/1
  Phase Ambiguity Corrector/2(validOut) -> validOut/1
  Delay9/1 -> syncPulseOut/1
  Delay8/1 -> Phase Ambiguity Corrector/1(dataIn)
  Average Estimates/1(avgEst) -> Phase Ambiguity Corrector/2(estimate)
  Delay7/1 -> Phase Ambiguity Corrector/3(validIn)
  Delay6/1 -> Delay10/1
  dataIn/1 -> Delay5/1
  validIn/1 -> Delay4/1
  Delay13/1 -> Delay8/1
  Phase Ambiguity Estimator/1(endOut) -> Average Estimates/1(endIn)
  Phase Ambiguity Estimator/3(validOut) -> Average Estimates/3(validIn)
  Delay12/1 -> Delay7/1
  Delay11/1 -> Delay6/1
  Phase Ambiguity Estimator/2(estOut) -> Average Estimates/2(estin)
  Delay/1 -> Delay13/1, EstDataLookback/1
  syncPulseIn/1 -> Phase Ambiguity Estimator/2(syncPulse), Delay3/1
  Delay2/1 -> Delay12/1, EstVldLookback/1
  Delay1/1 -> Delay11/1
  EstDataLookback/1 -> Phase Ambiguity Estimator/1(dataIn)
  EstVldLookback/1 -> Phase Ambiguity Estimator/3(validIn)

== system commhdlQPSKTxRxLoopback/Receiver/QPSK Rx/Frequency and Time Synchronizer/Preamble Detector ==
  dataIn : Inport
  validIn : Inport  Port=2
  Constant : Constant  Value=false  SampleTime=-1
  Correlator : Subsystem
  Delay : Delay  DelayLength=20
  Delay{1..5,11..14} (9 alike) : Delay  DelayLength=1
  Delay10 : Delay  DelayLength=searchSamples * 4
  Delay6 : Delay  DelayLength=6
  Delay7 : Delay  DelayLength=20
  Delay8 : Delay  DelayLength=6
  FIFO : Subsystem  mask{fifoSize=searchSamples, pushFullDiag=Error, popEmptyDiag=Error}
      mask prompts: fifoSize "FIFO size:"; pushFullDiag "Push full FIFO:"; popEmptyDiag "Pop empty FIFO:"
      mask TypeOptions pushFullDiag: Ignore | Warning | Error
      mask TypeOptions popEmptyDiag: Ignore | Warning | Error
  Logical Operator : Logic  AllPortsSameDT=off  OutDataTypeStr=boolean
  No HDL : Subsystem
  Peak Search : Subsystem  VariantControl=new  mask{samplesPerFrame=searchSamples}
      mask prompts: samplesPerFrame "Number of samples to search:"
      mask init:
      | samplesPerFrame1x            = samplesPerFrame;
      |     searchDuration               = samplesPerFrame1x;
  Relational Operator : RelationalOperator  Operator=>  OutDataTypeStr=boolean  InputSameDT=off
  Terminator : Terminator
  Terminator1 : Terminator
  Timing Adjust : Subsystem
  dataOut : Outport
  syncPulse : Outport  Port=2
  validOut : Outport  Port=3
  wires:
  Delay/1 -> Delay6/1
  validIn/1 -> Delay2/1
  dataIn/1 -> Delay1/1
  Relational Operator/1 -> Peak Search/2(thresholdExceeded)
  Peak Search/3(success) -> Logical Operator/2  "success"
  Peak Search/2(done) -> Logical Operator/1  "done"
  Delay7/1 -> Delay8/1
  Timing Adjust/1(dataOut) -> Delay3/1  "synchronizedData"
  Timing Adjust/3(SyncPulse) -> Delay4/1  "synchronizedPulse"
  Timing Adjust/2(validOut) -> Delay5/1  "synchronizedValid"
  Delay3/1 -> dataOut/1
  Delay5/1 -> validOut/1
  Delay4/1 -> syncPulse/1
  Peak Search/1(timingOffset) -> Delay11/1
  Logical Operator/1 -> Delay12/1
  Delay10/1 -> FIFO/3(pop), Delay14/1
  Correlator/3(validOut) -> Peak Search/3(validIn), No HDL/Enable
  Correlator/2(threshold) -> Relational Operator/2, No HDL/2(In2)
  Correlator/1(dataOut) -> Relational Operator/1, Peak Search/1(corr), No HDL/1(In1)
  Delay8/1 -> FIFO/2(push), Delay10/1
  Delay1/1 -> Delay/1, Correlator/1(dataIn)
  Delay2/1 -> Delay7/1, Correlator/2(validIn)
  Delay11/1 -> Timing Adjust/1(timingOffset)
  Delay12/1 -> Timing Adjust/2(timingOffsetValid)
  Delay13/1 -> Timing Adjust/3(dataIn)
  Delay14/1 -> Timing Adjust/4(validIn)
  FIFO/2(numEntries) -> Terminator/1
  Constant/1 -> FIFO/4(reset)
  FIFO/3(validPop) -> Terminator1/1
  Delay6/1 -> FIFO/1(in)
  FIFO/1(out) -> Delay13/1

== system commhdlQPSKTxRxLoopback/Receiver/QPSK Rx/Frequency and Time Synchronizer/Symbol Synchronizer ==
  dataIn : Inport
  validIn : Inport  Port=2
  Data Type Conversion4 : DataTypeConversion  OutDataTypeStr=fixdt(1,16,14)  SaturateOnIntegerOverflow=off  RndMeth=Floor
  Delay{1..4,6,8..9} (7 alike) : Delay  DelayLength=1
  Delay5 : Delay  DelayLength=12
  Delay7 : Delay  DelayLength=12
  Gardner TED : Subsystem
  Integer Delay{1..4} (4 alike) : Delay  DelayLength=1
  Interpolation Control : MATLAB Function
  Interpolation Filter : Subsystem
  Loop Filter : Subsystem
  No HDL : Subsystem
  Rate Handle : Subsystem
  dataOut : Outport
  validOut : Outport  Port=2
  wires:
  Loop Filter/1(v) -> Delay4/1
  Gardner TED/1(e) -> Delay3/1
  Interpolation Control/2(Underflow) -> Integer Delay3/1
  Integer Delay4/1 -> Interpolation Filter/2(mu)
  dataIn/1 -> No HDL/1(data), Integer Delay1/1
  Integer Delay3/1 -> Delay5/1
  Delay3/1 -> Loop Filter/1(e)
  Delay4/1 -> Interpolation Control/1(Delta)
  Data Type Conversion4/1 -> Rate Handle/1(dataIn)
  Delay1/1 -> Data Type Conversion4/1
  Delay6/1 -> Rate Handle/3(validIn)
  Delay7/1 -> Delay6/1
  validIn/1 -> No HDL/2(valid), Integer Delay2/1
  Rate Handle/2(validOut) -> validOut/1
  Rate Handle/1(dataOut) -> dataOut/1
  Interpolation Filter/1(interpolant) -> Delay8/1, Delay1/1
  Interpolation Control/1(mu) -> Integer Delay4/1
  Delay2/1 -> Rate Handle/2(strobe)
  Delay5/1 -> Delay9/1, Delay2/1
  Integer Delay1/1 -> Interpolation Filter/1(In)
  Integer Delay2/1 -> Delay7/1
  Delay8/1 -> Gardner TED/1(data)
  Delay9/1 -> Gardner TED/2(strobe)

== system commhdlQPSKTxRxLoopback/Receiver/QPSK Rx/QPSK Demodulator/Serializer ==
  u : Inport
  In2 : Inport  Port=2
  Delay1 : Delay  DelayLength=1
  Delay4 : Delay  DelayLength=1
  Demux : Demux  Outputs=2
  HDL Counter : hdlsllib/Sources/HDL Counter  CountType=Count limited  CountInit=0  CountStep=1  CountMax=1  CountFromType=Initial value  CountFrom=0  CountResetPort=off  CountLoadPort=off  CountEnbPort=on  CountDirPort=off  CountHitOutputPort=off  CountDataType=Unsigned  CountWordLen=1  CountFracLen=0  CountSampTime=1
  Logical Operator : Logic  Operator=OR  AllPortsSameDT=off  OutDataTypeStr=boolean
  Multiport Switch : MultiPortSwitch  DataPortOrder=Zero-based contiguous  Inputs=2  zeroidx=on  SaturateOnIntegerOverflow=off  InputSameDT=off
  Unit Delay Enabled Synchronous : hdlsllib/Discrete/Unit Delay Enabled Synchronous  InitialCondition=0.0  SampleTime=-1
  Out1 : Outport
  Out2 : Outport  Port=2
  wires:
  Demux/2 -> Multiport Switch/3
  Logical Operator/1 -> Out2/1, HDL Counter/1
  In2/1 -> Unit Delay Enabled Synchronous/2, Delay1/1
  HDL Counter/1 -> Multiport Switch/1
  Delay4/1 -> Logical Operator/2
  u/1 -> Unit Delay Enabled Synchronous/1
  Multiport Switch/1 -> Out1/1
  Demux/1 -> Multiport Switch/2
  Delay1/1 -> Logical Operator/1, Delay4/1
  Unit Delay Enabled Synchronous/1 -> Demux/1

== system commhdlQPSKTxRxLoopback/Transmitter/QPSK Tx/Bit Packetizer/Data Bits FIFO ==
  data : Inport
  push : Inport  Port=2
  Compare To Constant : simulink/Logic and Bit Operations/Compare To Constant  relop=>=  const=length(Preamble)  OutDataTypeStr=boolean
  Compare To Constant1 : simulink/Logic and Bit Operations/Compare To Constant  relop===  const=0  OutDataTypeStr=boolean
  Compare To Constant2 : simulink/Logic and Bit Operations/Compare To Constant  relop=~=  const=0  OutDataTypeStr=boolean
  Compare To Constant3 : simulink/Logic and Bit Operations/Compare To Constant  relop===  const=0  OutDataTypeStr=boolean
  Compare To Constant4 : simulink/Logic and Bit Operations/Compare To Constant  relop===  const=bitsPerPacket - 1  OutDataTypeStr=boolean
  Compare To Constant5 : hdlsllib/Logic and Bit Operations/Compare To Constant  relop=>=  const=Config.SamplesPerSymbol/2 -1  OutDataTypeStr=boolean
  Constant : Constant  Value=true  SampleTime=1/(Rsym*SamplesPerSymbol)
  Delay{1..7} (7 alike) : Delay  DelayLength=1
  HDL Counter : hdlsllib/Sources/HDL Counter  CountType=Count limited  CountInit=0  CountStep=1  CountMax=dataBitsPerPacket*2 - 1  CountFromType=Initial value  CountFrom=0  CountResetPort=off  CountLoadPort=off  CountEnbPort=on  CountDirPort=off  CountHitOutputPort=off  CountDataType=Unsigned  CountWordLen=nextpow2(dataBitsPerPacket*2 - 1)  CountFracLen=0  CountSampTime=1
  HDL Counter1 : hdlsllib/Sources/HDL Counter  CountType=Count limited  CountInit=0  CountStep=1  CountMax=dataBitsPerPacket*2 - 1  CountFromType=Initial value  CountFrom=0  CountResetPort=off  CountLoadPort=off  CountEnbPort=on  CountDirPort=off  CountHitOutputPort=off  CountDataType=Unsigned  CountWordLen=nextpow2(dataBitsPerPacket*2 - 1)  CountFracLen=0  CountSampTime=1
  HDL Counter2 : hdlsllib/Sources/HDL Counter  CountType=Count limited  CountInit=0  CountStep=1  CountMax=bitsPerPacket - 1  CountFromType=Initial value  CountFrom=0  CountResetPort=off  CountLoadPort=off  CountEnbPort=on  CountDirPort=off  CountHitOutputPort=off  CountDataType=Unsigned  CountWordLen=nextpow2(bitsPerPacket)  CountFracLen=0  CountSampTime=1
  HDL Counter3 : hdlsllib/Sources/HDL Counter  CountType=Count limited  CountInit=0  CountStep=1  CountMax=max(1, Config.SamplesPerSymbol/2 -1)  CountFromType=Initial value  CountFrom=0  CountResetPort=off  CountLoadPort=off  CountEnbPort=on  CountDirPort=off  CountHitOutputPort=off  CountDataType=Unsigned  CountWordLen=max(1, nextpow2(Config.SamplesPerSymbol/2))  CountFracLen=0  CountSampTime=1
  Logical Operator : Logic  Inputs=3  AllPortsSameDT=off  OutDataTypeStr=boolean
  Logical Operator1 : Logic  Inputs=3  AllPortsSameDT=off  OutDataTypeStr=boolean
  MATLAB Function1 : MATLAB Function  TreatAsAtomicUnit=on
  No HDL : Subsystem
  RAM Frame Status Indicator : MATLAB Function  TreatAsAtomicUnit=on
  Simple Dual Port RAM : hdlsllib/HDL RAMs/Simple Dual Port RAM  ram_size=nextpow2(dataBitsPerPacket*2 - 1)
  Unit Delay Enabled Resettable Synchronous : hdlsllib/Discrete/Unit Delay Enabled Resettable Synchronous  InitialCondition=0.0  SampleTime=-1
  dataOut : Outport
  activeFrame : Outport  Port=2
  sampleCount : Outport  Port=3
  sampleCountValid : Outport  Port=4
  fullRAM : Outport  Port=5
  wires:
  HDL Counter1/1 -> Simple Dual Port RAM/4
  HDL Counter/1 -> Simple Dual Port RAM/2
  data/1 -> Simple Dual Port RAM/1
  Constant/1 -> HDL Counter3/1
  HDL Counter2/1 -> Compare To Constant/1, Delay2/1, Compare To Constant3/1
  Compare To Constant1/1 -> Unit Delay Enabled Resettable Synchronous/3
  RAM Frame Status Indicator/1(out) -> Delay3/1
  Compare To Constant2/1 -> Logical Operator1/1, Unit Delay Enabled Resettable Synchronous/1
  Compare To Constant3/1 -> Unit Delay Enabled Resettable Synchronous/2
  Compare To Constant/1 -> Delay1/1
  Delay1/1 -> Logical Operator/2
  Delay2/1 -> Delay5/1
  Delay3/1 -> Compare To Constant2/1, Compare To Constant1/1
  Simple Dual Port RAM/1 -> dataOut/1
  Delay4/1 -> Logical Operator/3, Delay6/1
  Delay5/1 -> Compare To Constant4/1, sampleCount/1
  Delay6/1 -> Logical Operator1/3, sampleCountValid/1
  Unit Delay Enabled Resettable Synchronous/1 -> Logical Operator/1
  Compare To Constant4/1 -> Logical Operator1/2
  Logical Operator1/1 -> activeFrame/1
  Logical Operator/1 -> RAM Frame Status Indicator/2(pop), MATLAB Function1/2(rd), No HDL/2(pop), HDL Counter1/1
  push/1 -> MATLAB Function1/1(wr), RAM Frame Status Indicator/1(push), No HDL/1(push), HDL Counter/1, Simple Dual Port RAM/3
  MATLAB Function1/1(full) -> Delay7/1
  Delay7/1 -> fullRAM/1
  HDL Counter3/1 -> Compare To Constant5/1
  Compare To Constant5/1 -> HDL Counter2/1, Delay4/1
